simulink model "ECU1119_18b_st"  (R2018b)
settings: Solver=FixedStepDiscrete  StartTime=0.0  StopTime=10.0  RelTol=1e-3
InitFcn:
  | mbd_mpc_consistency_checks(bdroot(gcs));
values from neighbouring files (symbols this model uses):
  ANRtarget = 1.05    [Engine_init.m]
  EGRKi = 0.03    [Engine_init.m]
  EGRKp = 1.2*3    (= 3.6)    [Engine_init.m]
  EGRMax = 1    [Engine_init.m]
  EGRMin = 0    [Engine_init.m]
  EGRTgt = [0.25,0.22,0.20,0.18,0.16,0.12,0.10 ... (first row only)    [Engine_init.m]
  EGRTgt_x = [700,1200,1400,1600,1800,2000,2200]    [Engine_init.m]
  EGRTgt_y = [20,60,100,140,160]    [Engine_init.m]
  EngineSpdTgt = [700:150:2200]    [Engine_init.m]
  EngineSpdTgt_x = [0:10:100]    [Engine_init.m]
  FuelCyleMax = [40,50,60,60,60 ... (first row only)    [Engine_init.m]
  FuelCyleMax_x = [120,180,240,300,360]    [Engine_init.m]
  FuelCyleMax_y = [700,1200,1400,1600,1800,2000,2200]    [Engine_init.m]
  FuelCyleMaxSw = 0    [Engine_init.m]
  FuelCyleMin = 10    [Engine_init.m]
  FuelKd = 0    [Engine_init.m]
  FuelKi = 0.009*5    (= 0.045)    [Engine_init.m]
  FuelKp = 0.03*5    (= 0.15)    [Engine_init.m]
  Regen_Enable_SW = true    [Engine_init.m]
  Soot_Load_Off = 4    [Engine_init.m]
  Soot_Load_On = 18    [Engine_init.m]
  T_regen_max = 680    [Engine_init.m]
  T_regen_min = 550    [Engine_init.m]
undefined symbols (not defined in the file or in its folder): fifo_0_vect, fifo_1_vect, LQFP, pts1_fifo_0_vect, pts1_fifo_1_vect, pts2_fifo_0_vect, pts2_fifo_1_vect, pts3_fifo_0_vect, pts3_fifo_1_vect, pts4_fifo_0_vect, pts4_fifo_1_vect
libraries: mbd_mpc574x_ec_toolbox x111, simulink x12, canmsglib x8
(part 2 of 5)

== system ECU1119_18b_st/ECU ==
  note: 改成%单位了
  EngineSpd_rpm : Inport
  EngineInfo : Inport  Port=2
  ThrottleCmd_pct : Inport  Port=3
  Bus Creator : BusCreator  Inputs=6
  Bus Selector : BusSelector  OutputSignals=Obj_Fast_Fb1 (signal 1).FuelCycle_Act_mg,Obj_Fast_Fb1 (signal 1).EGR_Ratio_Act,Obj_Fast_Fb1 (signal 2).RailPrs_kpa,Obj_Fast_Fb1 (signal 2).IntakeMass_kgph,Obj_Temp_Fb1 (signal 3).DOC_In_Temp_C,Obj_Temp_Fb1 (signal 3).DOC_Out_Temp_C,Obj_Temp_Fb1 (signal 3).DPF_Out_Temp_C,Obj_Temp_Fb2 (signal 4).SCR_Out_Temp_C,Obj_Temp_Fb2 (signal 4).ExhMassFlow_kgph,Obj_Slow_Fb1 (signal 5).NOx_SCR_In_gph,Obj_Slow_Fb1 (signal 5).NOx_SCR_Out_gph,Obj_Slow_Fb1 (signal 5).SootLoad_g,Obj_Slow_Fb1 (signal 5).DPF_dP_kPa,Obj_Slow_Fb2 (signal 6).NH3_Store_g,Obj_Slow_Fb2 (signal 6).O2_frac_pct
  ECU : Subsystem
  Gain{,1..4} (5 alike) : Gain
  EngineCmd : Outport  VectorParamsAs1DForOutWhenUnconnected=on
  wires:
  Bus Selector/13 -> ECU/14(DPF_DP)  "<DPF_dP_kPa>"
  Bus Selector/1 -> ECU/2(FuleCyle_mg)  "<FuelCycle_Act_mg>"
  Bus Selector/14 -> Gain3/1  "<NH3_Store_g>"
  Bus Selector/9 -> ECU/10(ExhMassFlow)  "<ExhMassFlow_kgph>"
  Bus Selector/3 -> ECU/4(RailPrs_kpa)  "<RailPrs_kpa>"
  EngineInfo/1 -> Bus Selector/1
  Bus Selector/10 -> ECU/11(mNOx_SCR_in)  "<NOx_SCR_In_gph>"
  Bus Selector/11 -> Gain2/1  "<NOx_SCR_Out_gph>"
  Bus Selector/12 -> ECU/13(DPF_SootLoad)  "<SootLoad_g>"
  Bus Selector/15 -> Gain4/1  "<O2_frac_pct>"
  Bus Selector/2 -> ECU/3(EGRRatio)  "<EGR_Ratio_Act>"
  Bus Selector/5 -> Gain/1  "<DOC_In_Temp_C>"
  Bus Selector/4 -> ECU/5(IntakeMass)  "<IntakeMass_kgph>"
  Bus Selector/6 -> ECU/7(ExhTemp_DOC_out)  "<DOC_Out_Temp_C>"
  Bus Selector/7 -> ECU/8(ExhTemp_DPF_out)  "<DPF_Out_Temp_C>"
  Bus Selector/8 -> Gain1/1  "<SCR_Out_Temp_C>"
  ECU/3(EGROpeningTgt_pct) -> Bus Creator/3  "EGROpeningTgt_pct"
  ECU/2(FuelCyleTgt_mg) -> Bus Creator/2  "FuelCyleTgt_mg"
  ECU/6(mUREA_target) -> Bus Creator/6  "mUREA_target"
  ECU/1(EngineSpdTgt_rpm) -> Bus Creator/1  "EngineSpdTgt_rpm"
  ECU/5(DPF_regen_req) -> Bus Creator/5  "DPF_regen_req"
  ECU/4(PostInj_Request) -> Bus Creator/4  "PostInj_Request"
  EngineSpd_rpm/1 -> ECU/1(EngineSpd_rpm)
  Bus Creator/1 -> EngineCmd/1
  ThrottleCmd_pct/1 -> ECU/17(ThrottleCmd_pct)
  Gain/1 -> ECU/6(ExhTemp_DOC_in)
  Gain1/1 -> ECU/9(ExhTemp_SCR_out)
  Gain2/1 -> ECU/12(mNOx_SCR_out)
  Gain3/1 -> ECU/15(NH3_Store)
  Gain4/1 -> ECU/16(O2_frac)

== system ECU1119_18b_st/GPIO  ==
  note: LS
  note: PWM
  note: HS
  ETC : Subsystem
  HS : Subsystem
  PWM_OUT : Subsystem  Commented=on
  SPI0: LS09_14_15_16_1_2_11_4 : Subsystem
  SPI3: LS03_06_07_08_10_12_13_17_18_19 : Subsystem

== system ECU1119_18b_st/Init ==
  CAN_init : Subsystem
  Data Store Read1 : DataStoreRead  DataStoreName=VCU_Mode
  Data Store Read3 : DataStoreRead  DataStoreName=Init_flg
  If1 : If  IfExpression=u1 == 2  ShowElse=off
  If2 : If  IfExpression=u1 == 0  ShowElse=off
  Init : Subsystem
  wires:
  Data Store Read3/1 -> If2/1
  If2/1 -> Init/Action
  Data Store Read1/1 -> If1/1
  If1/1 -> CAN_init/Action

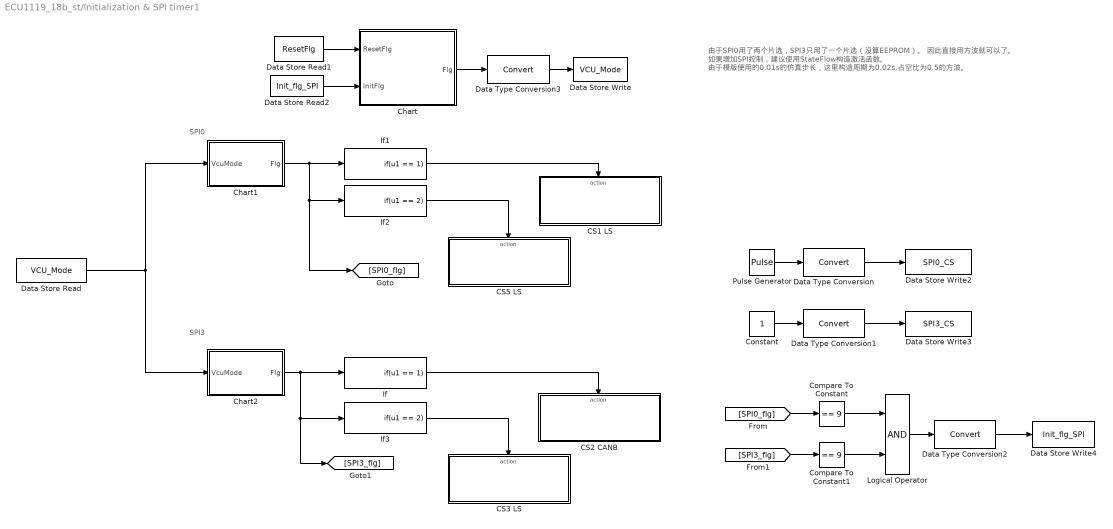
== system ECU1119_18b_st/Initialization & SPI timer1 ==
  note: 由于SPI0用了两个片选，SPI3只用了一个片选（没算EEPROM）。
      | 因此直接用方波就可以了。
      | 如果增加SPI控制，建议使用StateFlow构造激活函数。
      | 由于模版使用的0.01s的仿真步长，这里构造周期为0.02s,占空比为0.5的方波。
  note: SPI3
  note: SPI0
  CS1 LS : Subsystem
  CS2 CANB : Subsystem
  CS3 LS : Subsystem
  CS5 LS : Subsystem
  Chart : Stateflow chart  TreatAsAtomicUnit=on
  Chart1 : Stateflow chart  TreatAsAtomicUnit=on
  Chart2 : Stateflow chart  TreatAsAtomicUnit=on
  Compare To Constant : simulink/Logic and Bit Operations/Compare To Constant  relop===  const=9  OutDataTypeStr=boolean
  Compare To Constant1 : simulink/Logic and Bit Operations/Compare To Constant  relop===  const=9  OutDataTypeStr=boolean
  Constant : Constant
  Data Store Read : DataStoreRead  DataStoreName=VCU_Mode
  Data Store Read1 : DataStoreRead  DataStoreName=ResetFlg
  Data Store Read2 : DataStoreRead  DataStoreName=Init_flg_SPI
  Data Store Write : DataStoreWrite  DataStoreName=VCU_Mode
  Data Store Write2 : DataStoreWrite  DataStoreName=SPI0_CS
  Data Store Write3 : DataStoreWrite  DataStoreName=SPI3_CS
  Data Store Write4 : DataStoreWrite  DataStoreName=Init_flg_SPI
  Data Type Conversion{,1..3} (4 alike) : DataTypeConversion
  If : If  IfExpression=u1 == 1  ShowElse=off
  If1 : If  IfExpression=u1 == 1  ShowElse=off
  If2 : If  IfExpression=u1 == 2  ShowElse=off
  If3 : If  IfExpression=u1 == 2  ShowElse=off
  Logical Operator : Logic  AllPortsSameDT=off  OutDataTypeStr=boolean
  Pulse Generator : DiscretePulseGenerator  PulseType=Time based  Period=0.01  PulseWidth=50
  wires:
  If/1 -> CS2 CANB/Action
  Chart/1(Flg) -> Data Type Conversion3/1
  Data Store Read2/1 -> Chart/2(InitFlg)
  If1/1 -> CS1 LS/Action
  Chart2/1(Flg) -> If3/1, [SPI3_flg], If/1
  Data Store Read/1 -> Chart2/1(VcuMode), Chart1/1(VcuMode)
  If2/1 -> CS5 LS/Action
  [SPI0_flg] -> Compare To Constant/1
  [SPI3_flg] -> Compare To Constant1/1
  Compare To Constant/1 -> Logical Operator/1
  Compare To Constant1/1 -> Logical Operator/2
  Logical Operator/1 -> Data Type Conversion2/1
  If3/1 -> CS3 LS/Action
  Pulse Generator/1 -> Data Type Conversion/1
  Constant/1 -> Data Type Conversion1/1
  Data Type Conversion/1 -> Data Store Write2/1
  Data Type Conversion1/1 -> Data Store Write3/1
  Data Type Conversion2/1 -> Data Store Write4/1
  Data Type Conversion3/1 -> Data Store Write/1
  Chart1/1(Flg) -> If1/1, [SPI0_flg], If2/1
  Data Store Read1/1 -> Chart/1(ResetFlg)

== system ECU1119_18b_st/Power Managment ==
  PowerMode : Inport
  Data Type Conversion : DataTypeConversion
  HS1 : mbd_mpc574x_ec_toolbox/GPIO Blocks/Digital_Output  Priority=1  gpio_pin=PTF6: [SIUL2_GPIO86 | General Purpose IO PF[6]]  gpio_drive_strength=Disabled
      settings: SourceProductName=NXP Model-Based Design Toolbox for MPC57xx MCUs
  HS4 : mbd_mpc574x_ec_toolbox/GPIO Blocks/Digital_Output  Priority=1  gpio_pin=PTA13: [SIUL2_GPIO13 | General Purpose IO PA[13]]  gpio_drive_strength=Disabled
      settings: SourceProductName=NXP Model-Based Design Toolbox for MPC57xx MCUs
  wires:
  PowerMode/1 -> Data Type Conversion/1
  Data Type Conversion/1 -> HS4/1, HS1/1

== system ECU1119_18b_st/SPI_EEPROM ==
  Data Store Memory : DataStoreMemory  DataStoreName=A_write  ReadBeforeWriteMsg=warning  WriteAfterWriteMsg=warning  WriteAfterReadMsg=warning  ShowAdditionalParam=off  OutDataTypeStr=single
      settings: RTWStateStorageClass=ExportedGlobal
  Data Store Memory10 : DataStoreMemory  DataStoreName=A_read  ReadBeforeWriteMsg=warning  WriteAfterWriteMsg=warning  WriteAfterReadMsg=warning  ShowAdditionalParam=off  OutDataTypeStr=single
      settings: RTWStateStorageClass=ExportedGlobal
  Data Store Memory18 : DataStoreMemory  DataStoreName=SPI0_CTRL0  ReadBeforeWriteMsg=warning  WriteAfterWriteMsg=warning  WriteAfterReadMsg=warning  ShowAdditionalParam=off  OutDataTypeStr=uint8
      settings: RTWStateStorageClass=ExportedGlobal
  Data Store Read : DataStoreRead  DataStoreName=SPI0_CTRL0
  SPI_read : Subsystem  TreatAsAtomicUnit=on
  SPI_write : Subsystem  TreatAsAtomicUnit=on
  Switch Case : SwitchCase  CaseConditions={1,2}  ShowDefaultCase=off
  wires:
  Data Store Read/1 -> Switch Case/1
  Switch Case/2 -> SPI_write/Action
  Switch Case/1 -> SPI_read/Action

== system ECU1119_18b_st/SigIn ==
  note: CAN2
  note: HardWareSignalIn
  AI : Subsystem  Commented=on
  CAN0_Rx_500 : mbd_mpc574x_ec_toolbox/Communication Blocks/CAN Blocks/FCAN_Isr  can_instance=2  can_event=Rx Complete
      settings: SourceProductName=NXP Model-Based Design Toolbox for MPC57xx MCUs
  CAN2 : Subsystem  TreatAsAtomicUnit=on
      settings: RTWSystemCode=Nonreusable function
  DI : Subsystem  Commented=on
  PWM : Subsystem  Commented=on
  Terminator : Terminator  Commented=on
  Terminator3 : Terminator  Commented=on
  Terminator5 : Terminator  Commented=on
  Terminator8 : Terminator
  EngineSpd_rpm : Outport  VectorParamsAs1DForOutWhenUnconnected=on
  EngineInfo : Outport  Port=2  VectorParamsAs1DForOutWhenUnconnected=on
  ThrottleCmd_pct : Outport  Port=3  VectorParamsAs1DForOutWhenUnconnected=on
  wires:
  CAN0_Rx_500/5 -> CAN2/3(length)
  CAN0_Rx_500/3 -> CAN2/1(ID)
  CAN0_Rx_500/4 -> CAN2/2(Data)
  CAN0_Rx_500/6 -> CAN2/4(timestamp)
  CAN0_Rx_500/1 -> CAN2/Trigger
  CAN0_Rx_500/2 -> Terminator8/1
  PWM/1(PWMIn) -> Terminator/1
  DI/1(DI) -> Terminator3/1
  AI/1(AI) -> Terminator5/1
  CAN2/3(ThrottleCmd_pct) -> ThrottleCmd_pct/1
  CAN2/2(EngineInfo) -> EngineInfo/1
  CAN2/1(EngineSpd_rpm) -> EngineSpd_rpm/1

== system ECU1119_18b_st/SigOut ==
  note: 10ms
  note: 100ms
  EngCmd : Inport
  Pulse Generator : DiscretePulseGenerator  PulseType=Time based  Period=0.1  PulseWidth=5
  Pulse Generator1 : DiscretePulseGenerator  PulseType=Time based  Period=0.01  PulseWidth=50
  Rate Transition : RateTransition
  Rate Transition1 : RateTransition
  VCU_Cmd_Fast : Subsystem  TreatAsAtomicUnit=on  SystemSampleTime=0.01
  VCU_Cmd_Slow : Subsystem  TreatAsAtomicUnit=on  SystemSampleTime=0.01
  wires:
  EngCmd/1 -> Rate Transition1/1, Rate Transition/1
  Rate Transition/1 -> VCU_Cmd_Fast/1("EngCmd ")
  Pulse Generator1/1 -> VCU_Cmd_Fast/Trigger
  Pulse Generator/1 -> VCU_Cmd_Slow/Trigger
  Rate Transition1/1 -> VCU_Cmd_Slow/1("EngCmd ")

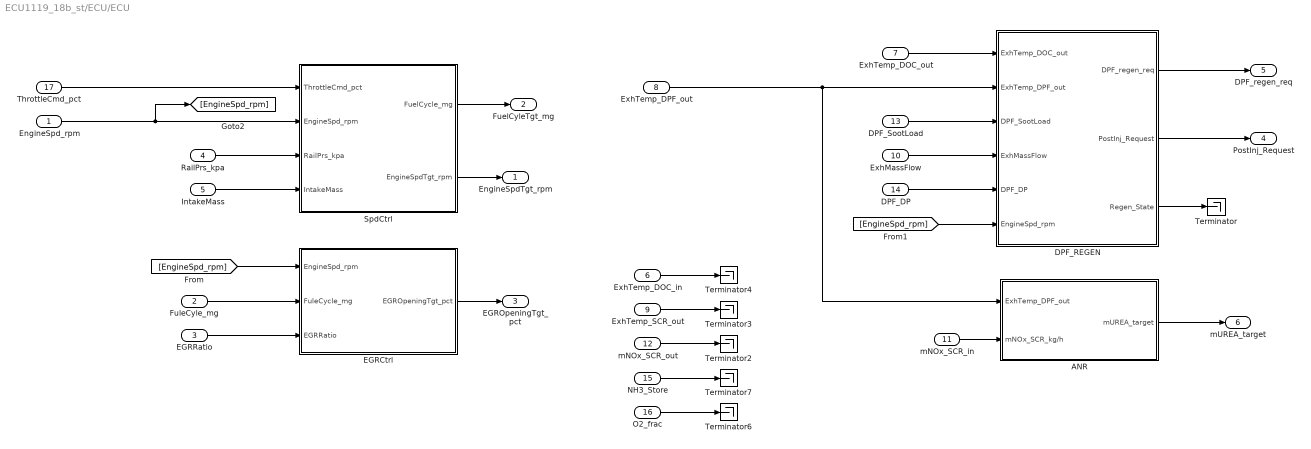
== system ECU1119_18b_st/ECU/ECU ==
  EngineSpd_rpm : Inport
  FuleCyle_mg : Inport  Port=2
  EGRRatio : Inport  Port=3
  RailPrs_kpa : Inport  Port=4
  IntakeMass : Inport  Port=5
  ExhTemp_DOC_in : Inport  Port=6
  ExhTemp_DOC_out : Inport  Port=7
  ExhTemp_DPF_out : Inport  Port=8
  ExhTemp_SCR_out : Inport  Port=9
  ExhMassFlow : Inport  Port=10
  mNOx_SCR_in : Inport  Port=11
  mNOx_SCR_out : Inport  Port=12
  DPF_SootLoad : Inport  Port=13
  DPF_DP : Inport  Port=14
  NH3_Store : Inport  Port=15
  O2_frac : Inport  Port=16
  ThrottleCmd_pct : Inport  Port=17
  ANR : Subsystem
  DPF_REGEN : Subsystem
  EGRCtrl : Subsystem
  SpdCtrl : Subsystem
  Terminator{,2..4,6..7} (6 alike) : Terminator
  EngineSpdTgt_rpm : Outport  VectorParamsAs1DForOutWhenUnconnected=on
  FuelCyleTgt_mg : Outport  Port=2  VectorParamsAs1DForOutWhenUnconnected=on
  EGROpeningTgt_pct : Outport  Port=3  VectorParamsAs1DForOutWhenUnconnected=on
  PostInj_Request : Outport  Port=4  VectorParamsAs1DForOutWhenUnconnected=on
  DPF_regen_req : Outport  Port=5  VectorParamsAs1DForOutWhenUnconnected=on
  mUREA_target : Outport  Port=6  VectorParamsAs1DForOutWhenUnconnected=on
  wires:
  SpdCtrl/1(FuelCycle_mg) -> FuelCyleTgt_mg/1
  EngineSpd_rpm/1 -> [EngineSpd_rpm], SpdCtrl/2(EngineSpd_rpm)
  FuleCyle_mg/1 -> EGRCtrl/2(FuleCycle_mg)
  EGRCtrl/1(EGROpeningTgt_pct) -> EGROpeningTgt_pct/1
  EGRRatio/1 -> EGRCtrl/3(EGRRatio)
  RailPrs_kpa/1 -> SpdCtrl/3(RailPrs_kpa)
  IntakeMass/1 -> SpdCtrl/4(IntakeMass)
  [EngineSpd_rpm] -> EGRCtrl/1(EngineSpd_rpm)
  mNOx_SCR_in/1 -> ANR/2(mNOx_SCR_kg/h)
  ANR/1(mUREA_target) -> mUREA_target/1
  ExhTemp_DPF_out/1 -> DPF_REGEN/2(ExhTemp_DPF_out), ANR/1(ExhTemp_DPF_out)
  DPF_SootLoad/1 -> DPF_REGEN/3(DPF_SootLoad)
  ExhMassFlow/1 -> DPF_REGEN/4(ExhMassFlow)
  DPF_REGEN/1(DPF_regen_req) -> DPF_regen_req/1
  ExhTemp_DOC_in/1 -> Terminator4/1
  mNOx_SCR_out/1 -> Terminator2/1
  ExhTemp_SCR_out/1 -> Terminator3/1
  NH3_Store/1 -> Terminator7/1
  O2_frac/1 -> Terminator6/1
  DPF_DP/1 -> DPF_REGEN/5(DPF_DP)
  ExhTemp_DOC_out/1 -> DPF_REGEN/1(ExhTemp_DOC_out)
  [EngineSpd_rpm] -> DPF_REGEN/6(EngineSpd_rpm)
  DPF_REGEN/2(PostInj_Request) -> PostInj_Request/1
  ThrottleCmd_pct/1 -> SpdCtrl/1(ThrottleCmd_pct)
  SpdCtrl/2(EngineSpdTgt_rpm) -> EngineSpdTgt_rpm/1
  DPF_REGEN/3(Regen_State) -> Terminator/1

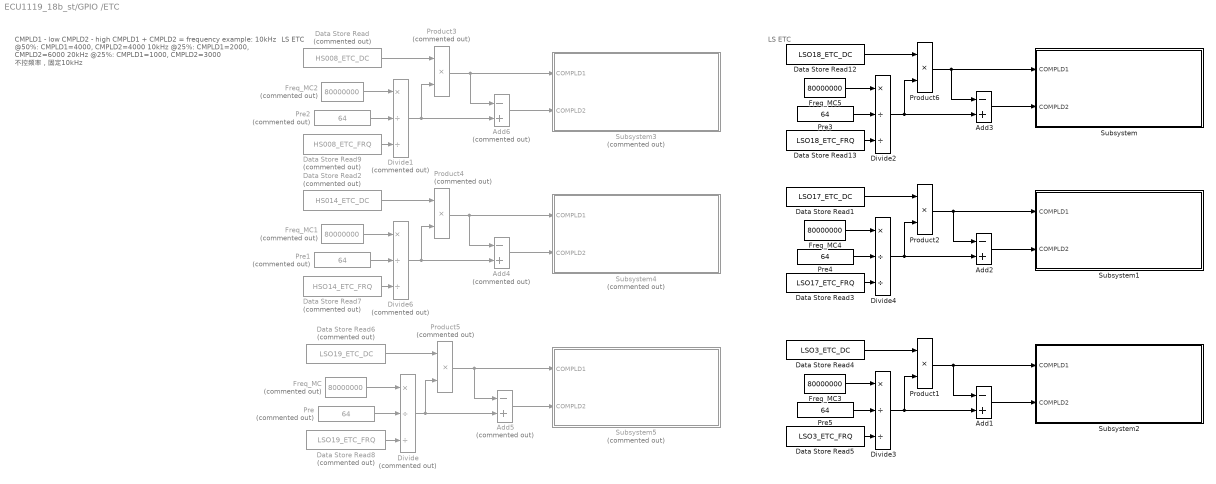
== system ECU1119_18b_st/GPIO /ETC ==
  note: CMPLD1 - low
      | CMPLD2 - high
      | CMPLD1 + CMPLD2 = frequency
      | example:
      | 10kHz @50%: CMPLD1=4000, CMPLD2=4000
      | 10kHz @25%: CMPLD1=2000, CMPLD2=6000
      | 20kHz @25%: CMPLD1=1000, CMPLD2=3000
      |
      | 不控频率，固定10kHz
  note: LS ETC
  note: LS ETC
  Add1 : Sum  Inputs=-+
  Add2 : Sum  Inputs=-+
  Add3 : Sum  Inputs=-+
  Add4 : Sum  Commented=on  Inputs=-+
  Add5 : Sum  Commented=on  Inputs=-+
  Add6 : Sum  Commented=on  Inputs=-+
  Data Store Read : DataStoreRead  Commented=on  DataStoreName=HS008_ETC_DC
  Data Store Read1 : DataStoreRead  DataStoreName=LSO17_ETC_DC
  Data Store Read12 : DataStoreRead  DataStoreName=LSO18_ETC_DC
  Data Store Read13 : DataStoreRead  DataStoreName=LSO18_ETC_FRQ
  Data Store Read2 : DataStoreRead  Commented=on  DataStoreName=HS014_ETC_DC
  Data Store Read3 : DataStoreRead  DataStoreName=LSO17_ETC_FRQ
  Data Store Read4 : DataStoreRead  DataStoreName=LSO3_ETC_DC
  Data Store Read5 : DataStoreRead  DataStoreName=LSO3_ETC_FRQ
  Data Store Read6 : DataStoreRead  Commented=on  DataStoreName=LSO19_ETC_DC
  Data Store Read7 : DataStoreRead  Commented=on  DataStoreName=HSO14_ETC_FRQ
  Data Store Read8 : DataStoreRead  Commented=on  DataStoreName=LSO19_ETC_FRQ
  Data Store Read9 : DataStoreRead  Commented=on  DataStoreName=HS008_ETC_FRQ
  Divide : Product  Commented=on  Inputs=*//
  Divide1 : Product  Commented=on  Inputs=*//
  Divide2 : Product  Inputs=*//
  Divide3 : Product  Inputs=*//
  Divide4 : Product  Inputs=*//
  Divide6 : Product  Commented=on  Inputs=*//
  Freq_MC : Constant  Commented=on  Value=80000000  OutDataTypeStr=single
  Freq_MC1 : Constant  Commented=on  Value=80000000  OutDataTypeStr=single
  Freq_MC2 : Constant  Commented=on  Value=80000000  OutDataTypeStr=single
  Freq_MC3 : Constant  Value=80000000  OutDataTypeStr=single
  Freq_MC4 : Constant  Value=80000000  OutDataTypeStr=single
  Freq_MC5 : Constant  Value=80000000  OutDataTypeStr=single
  Pre : Constant  Commented=on  Value=64
  Pre1 : Constant  Commented=on  Value=64
  Pre2 : Constant  Commented=on  Value=64
  Pre3 : Constant  Value=64
  Pre4 : Constant  Value=64
  Pre5 : Constant  Value=64
  Product1 : Product
  Product2 : Product
  Product3 : Product  Commented=on
  Product4 : Product  Commented=on
  Product5 : Product  Commented=on
  Product6 : Product
  Subsystem : Subsystem
  Subsystem1 : Subsystem
  Subsystem2 : Subsystem
  Subsystem3 : Subsystem  Commented=on
  Subsystem4 : Subsystem  Commented=on
  Subsystem5 : Subsystem  Commented=on
  wires:
  Data Store Read6/1 -> Product5/1
  Product5/1 -> Add5/1, Subsystem5/1(COMPLD1)
  Add5/1 -> Subsystem5/2(COMPLD2)
  Add4/1 -> Subsystem4/2(COMPLD2)
  Data Store Read8/1 -> Divide/3
  Data Store Read2/1 -> Product4/1
  Freq_MC/1 -> Divide/1
  Divide/1 -> Product5/2, Add5/2
  Divide6/1 -> Product4/2, Add4/2
  Freq_MC1/1 -> Divide6/1
  Data Store Read7/1 -> Divide6/3
  Product4/1 -> Add4/1, Subsystem4/1(COMPLD1)
  Divide1/1 -> Product3/2, Add6/2
  Freq_MC2/1 -> Divide1/1
  Data Store Read9/1 -> Divide1/3
  Product3/1 -> Add6/1, Subsystem3/1(COMPLD1)
  Data Store Read/1 -> Product3/1
  Add6/1 -> Subsystem3/2(COMPLD2)
  Divide3/1 -> Product1/2, Add1/2
  Freq_MC3/1 -> Divide3/1
  Data Store Read5/1 -> Divide3/3
  Product1/1 -> Add1/1, Subsystem2/1(COMPLD1)
  Divide4/1 -> Product2/2, Add2/2
  Freq_MC4/1 -> Divide4/1
  Data Store Read3/1 -> Divide4/3
  Product2/1 -> Add2/1, Subsystem1/1(COMPLD1)
  Divide2/1 -> Product6/2, Add3/2
  Freq_MC5/1 -> Divide2/1
  Data Store Read13/1 -> Divide2/3
  Product6/1 -> Add3/1, Subsystem/1(COMPLD1)
  Data Store Read1/1 -> Product2/1
  Data Store Read4/1 -> Product1/1
  Data Store Read12/1 -> Product6/1
  Add1/1 -> Subsystem2/2(COMPLD2)
  Add2/1 -> Subsystem1/2(COMPLD2)
  Add3/1 -> Subsystem/2(COMPLD2)
  Pre/1 -> Divide/2
  Pre1/1 -> Divide6/2
  Pre2/1 -> Divide1/2
  Pre3/1 -> Divide2/2
  Pre4/1 -> Divide4/2
  Pre5/1 -> Divide3/2

== system ECU1119_18b_st/GPIO /HS ==
  note: 3A/5A
  note: 1A/3A
  note: 0.5A/1A
  Data Store Read : DataStoreRead  DataStoreName=HS001
  Data Store Read2 : DataStoreRead  DataStoreName=HS007
  Data Store Read4 : DataStoreRead  DataStoreName=HS002
  Data Store Read5 : DataStoreRead  DataStoreName=HS003
  Data Store Read6 : DataStoreRead  DataStoreName=HS004
  Data Store Read7 : DataStoreRead  DataStoreName=HS005
  Data Store Read9 : DataStoreRead  DataStoreName=HS010
  HS001 : mbd_mpc574x_ec_toolbox/GPIO Blocks/Digital_Output  Priority=1  gpio_pin=PTF5: [SIUL2_GPIO85 | General Purpose IO PF[5]]  gpio_drive_strength=Disabled
      settings: SourceProductName=NXP Model-Based Design Toolbox for MPC57xx MCUs
  "HS002 " : mbd_mpc574x_ec_toolbox/GPIO Blocks/Digital_Output  Priority=1  gpio_pin=PTF4: [SIUL2_GPIO84 | General Purpose IO PF[4]]  gpio_drive_strength=Disabled
      settings: SourceProductName=NXP Model-Based Design Toolbox for MPC57xx MCUs
  HS003 : mbd_mpc574x_ec_toolbox/GPIO Blocks/Digital_Output  Priority=1  gpio_pin=PTF3: [SIUL2_GPIO83 | General Purpose IO PF[3]]  gpio_drive_strength=Disabled
      settings: SourceProductName=NXP Model-Based Design Toolbox for MPC57xx MCUs
  HS004 : mbd_mpc574x_ec_toolbox/GPIO Blocks/Digital_Output  Priority=1  gpio_pin=PTB6: [SIUL2_GPIO22 | General Purpose IO PB[6]]  gpio_drive_strength=Disabled
      settings: SourceProductName=NXP Model-Based Design Toolbox for MPC57xx MCUs
  HS005 : mbd_mpc574x_ec_toolbox/GPIO Blocks/Digital_Output  Priority=1  gpio_pin=PTA12: [SIUL2_GPIO12 | General Purpose IO PA[12]]  gpio_drive_strength=Disabled
      settings: SourceProductName=NXP Model-Based Design Toolbox for MPC57xx MCUs
  HS007 : mbd_mpc574x_ec_toolbox/GPIO Blocks/Digital_Output  Priority=1  gpio_pin=PTF7: [SIUL2_GPIO87 | General Purpose IO PF[7]]  gpio_drive_strength=Disabled
      settings: SourceProductName=NXP Model-Based Design Toolbox for MPC57xx MCUs
  HS010 : mbd_mpc574x_ec_toolbox/GPIO Blocks/Digital_Output  Priority=1  gpio_pin=PTF9: [SIUL2_GPIO89 | General Purpose IO PF[9]]  gpio_drive_strength=Disabled
      settings: SourceProductName=NXP Model-Based Design Toolbox for MPC57xx MCUs
  wires:
  Data Store Read/1 -> HS001/1
  Data Store Read5/1 -> HS003/1
  Data Store Read4/1 -> "HS002 "/1
  Data Store Read6/1 -> HS004/1
  Data Store Read7/1 -> HS005/1
  Data Store Read2/1 -> HS007/1
  Data Store Read9/1 -> HS010/1

== system ECU1119_18b_st/GPIO /PWM_OUT ==
  note: LS PWM
  note: HS PWM
  note: Example
  Data Store Read10 : DataStoreRead  DataStoreName=HSO14_PWM_DC
  Data Store Read11 : DataStoreRead  DataStoreName=HSO14_PWM_FRQ
  Data Store Read14 : DataStoreRead  DataStoreName=LSO19_PWM_DC
  Data Store Read15 : DataStoreRead  DataStoreName=LSO19_PWM_FRQ
  Data Store Read2 : DataStoreRead  DataStoreName=HSO08_PWM_DC
  Data Store Read9 : DataStoreRead  DataStoreName=HSO08_PWM_FRQ
  FreqCMD : Stateflow chart  Priority=0  Commented=on  TreatAsAtomicUnit=on
  PWM Configuration and Frequency Update : Subsystem  Commented=on
  PWM Configuration and Frequency Update1 : Subsystem
  PWM Configuration and Frequency Update4 : Subsystem
  wires:
  FreqCMD/1(freq) -> PWM Configuration and Frequency Update/1(In1)
  FreqCMD/2(dc) -> PWM Configuration and Frequency Update/2(In2)
  Data Store Read9/1 -> PWM Configuration and Frequency Update1/2(Fre A)
  Data Store Read2/1 -> PWM Configuration and Frequency Update1/1(PWM A)
  Data Store Read14/1 -> PWM Configuration and Frequency Update4/1(PWM A)
  Data Store Read10/1 -> PWM Configuration and Frequency Update1/3(PWM B)
  Data Store Read11/1 -> PWM Configuration and Frequency Update1/4(Fre B)
  Data Store Read15/1 -> PWM Configuration and Frequency Update4/2(Fre)

== system ECU1119_18b_st/GPIO /SPI0: LS09_14_15_16_1_2_11_4 ==
  note: 不要开，会重置SPI的初始化设置
  Compare To Constant : simulink/Logic and Bit Operations/Compare To Constant  relop===  const=2  OutDataTypeStr=boolean
  Constant : Constant  OutDataTypeStr=boolean
  Constant1 : Constant  OutDataTypeStr=boolean
  Constant2 : Constant  OutDataTypeStr=boolean
  Data Store Read : DataStoreRead  DataStoreName=VCU_Mode
  Data Store Read1 : DataStoreRead  DataStoreName=SPI0_CS
  LS_CTRL : Subsystem
  LS_CTRL1 : Subsystem
  LS_EN : mbd_mpc574x_ec_toolbox/GPIO Blocks/Digital_Output  Priority=1  gpio_pin=PTA2: [SIUL2_GPIO2 | General Purpose IO PA[2]]  gpio_drive_strength=Disabled
      settings: SourceProductName=NXP Model-Based Design Toolbox for MPC57xx MCUs
  LS_rst1 : mbd_mpc574x_ec_toolbox/GPIO Blocks/Digital_Output  Priority=1  gpio_pin=PTC10: [SIUL2_GPIO42 | General Purpose IO PC[10]]  gpio_drive_strength=Disabled
      settings: SourceProductName=NXP Model-Based Design Toolbox for MPC57xx MCUs
  LS_rst2 : mbd_mpc574x_ec_toolbox/GPIO Blocks/Digital_Output  Priority=1  gpio_pin=PTA1: [SIUL2_GPIO1 | General Purpose IO PA[1]]  gpio_drive_strength=Disabled
      settings: SourceProductName=NXP Model-Based Design Toolbox for MPC57xx MCUs
  Logical Operator : Logic  AllPortsSameDT=off  OutDataTypeStr=boolean
  Logical Operator1 : Logic  Operator=NOT  AllPortsSameDT=off  OutDataTypeStr=boolean
  wires:
  Constant1/1 -> LS_rst2/1
  Constant/1 -> LS_EN/1
  Constant2/1 -> LS_rst1/1
  Data Store Read/1 -> Compare To Constant/1
  Compare To Constant/1 -> Logical Operator/1
  Data Store Read1/1 -> Logical Operator/2
  Logical Operator/1 -> LS_CTRL1/Enable, Logical Operator1/1
  Logical Operator1/1 -> LS_CTRL/Enable

== system ECU1119_18b_st/GPIO /SPI3: LS03_06_07_08_10_12_13_17_18_19 ==
  Compare To Constant : simulink/Logic and Bit Operations/Compare To Constant  relop===  const=2  OutDataTypeStr=boolean
  Constant1 : Constant  OutDataTypeStr=boolean
  Constant3 : Constant  OutDataTypeStr=boolean
  Data Store Read : DataStoreRead  DataStoreName=VCU_Mode
  Data Store Read3 : DataStoreRead  DataStoreName=SPI3_CS
  LS_EN1 : mbd_mpc574x_ec_toolbox/GPIO Blocks/Digital_Output  Priority=1  gpio_pin=PTF10: [SIUL2_GPIO90 | General Purpose IO PF[10]]  gpio_drive_strength=Disabled
      settings: SourceProductName=NXP Model-Based Design Toolbox for MPC57xx MCUs
  LS_rst : mbd_mpc574x_ec_toolbox/GPIO Blocks/Digital_Output  Priority=1  gpio_pin=PTC14: [SIUL2_GPIO46 | General Purpose IO PC[14]]  gpio_drive_strength=Disabled
      settings: SourceProductName=NXP Model-Based Design Toolbox for MPC57xx MCUs
  Logical Operator : Logic  AllPortsSameDT=off  OutDataTypeStr=boolean
  Subsystem : Subsystem
  wires:
  Constant1/1 -> LS_EN1/1
  Constant3/1 -> LS_rst/1
  Data Store Read/1 -> Compare To Constant/1
  Data Store Read3/1 -> Logical Operator/2
  Compare To Constant/1 -> Logical Operator/1
  Logical Operator/1 -> Subsystem/Enable

== system ECU1119_18b_st/Init/CAN_init ==
  note: CAN2
  Action Port : ActionPort  ActionType=then
  Obj_Fast_Fb1 : mbd_mpc574x_ec_toolbox/Communication Blocks/CAN Blocks/FCAN_Receive  can_instance=2  can_mode=Non-blocking  can_timeout_ms=0  can_mb_idx=0  can_extended_id=off  can_is_remote=off  can_id=101  can_msg_mask=FFFFFFFF  show_adv_opts=off  can_use_rxfifo=off  can_fd_enable=off
      settings: SourceProductName=NXP Model-Based Design Toolbox for MPC57xx MCUs
  Obj_Fast_Fb2 : mbd_mpc574x_ec_toolbox/Communication Blocks/CAN Blocks/FCAN_Receive  can_instance=2  can_mode=Non-blocking  can_timeout_ms=0  can_mb_idx=1  can_extended_id=off  can_is_remote=off  can_id=102  can_msg_mask=FFFFFFFF  show_adv_opts=off  can_use_rxfifo=off  can_fd_enable=off
      settings: SourceProductName=NXP Model-Based Design Toolbox for MPC57xx MCUs
  Obj_Slow_Fb1 : mbd_mpc574x_ec_toolbox/Communication Blocks/CAN Blocks/FCAN_Receive  can_instance=2  can_mode=Non-blocking  can_timeout_ms=0  can_mb_idx=4  can_extended_id=off  can_is_remote=off  can_id=105  can_msg_mask=FFFFFFFF  show_adv_opts=off  can_use_rxfifo=off  can_fd_enable=off
      settings: SourceProductName=NXP Model-Based Design Toolbox for MPC57xx MCUs
  Obj_Slow_Fb2 : mbd_mpc574x_ec_toolbox/Communication Blocks/CAN Blocks/FCAN_Receive  can_instance=2  can_mode=Non-blocking  can_timeout_ms=0  can_mb_idx=5  can_extended_id=off  can_is_remote=off  can_id=106  can_msg_mask=FFFFFFFF  show_adv_opts=off  can_use_rxfifo=off  can_fd_enable=off
      settings: SourceProductName=NXP Model-Based Design Toolbox for MPC57xx MCUs
  Obj_Temp_Fb1 : mbd_mpc574x_ec_toolbox/Communication Blocks/CAN Blocks/FCAN_Receive  can_instance=2  can_mode=Non-blocking  can_timeout_ms=0  can_mb_idx=2  can_extended_id=off  can_is_remote=off  can_id=103  can_msg_mask=FFFFFFFF  show_adv_opts=off  can_use_rxfifo=off  can_fd_enable=off
      settings: SourceProductName=NXP Model-Based Design Toolbox for MPC57xx MCUs
  Obj_Temp_Fb2 : mbd_mpc574x_ec_toolbox/Communication Blocks/CAN Blocks/FCAN_Receive  can_instance=2  can_mode=Non-blocking  can_timeout_ms=0  can_mb_idx=3  can_extended_id=off  can_is_remote=off  can_id=104  can_msg_mask=FFFFFFFF  show_adv_opts=off  can_use_rxfifo=off  can_fd_enable=off
      settings: SourceProductName=NXP Model-Based Design Toolbox for MPC57xx MCUs

== system ECU1119_18b_st/Init/Init ==
  note: MainRelay
  Action Port : ActionPort  ActionType=then
  Chart : Stateflow chart  TreatAsAtomicUnit=on
  Constant : Constant
  Data Store Read1 : DataStoreRead  DataStoreName=KeyOn
  Data Store Write : DataStoreWrite  DataStoreName=LS001
  Data Store Write3 : DataStoreWrite  DataStoreName=Init_flg
  Data Type Conversion : DataTypeConversion
  Data Type Conversion1 : DataTypeConversion  OutDataTypeStr=boolean
  wires:
  Constant/1 -> Data Type Conversion/1
  Data Type Conversion/1 -> Data Store Write3/1
  Chart/1(LS001) -> Data Type Conversion1/1
  Data Store Read1/1 -> Chart/1(KeyOn)
  Data Type Conversion1/1 -> Data Store Write/1

== system ECU1119_18b_st/Initialization & SPI timer1/CS1 LS ==
  Action Port : ActionPort  ActionType=then
  Chart : Stateflow chart  TreatAsAtomicUnit=on
  Data Type Conversion{,1,3..4} (4 alike) : DataTypeConversion
  Demux1 : Demux  Outputs=2
  SPI_Master_Transfer_To1 : mbd_mpc574x_ec_toolbox/Communication Blocks/SPI Blocks/SPI_Master_Transfer  Priority=2  InstanceNumber=0  xfermode=Non blocking  timeout=50  spi_upd=on  WhichPCS=5
      settings: SourceProductName=NXP Model-Based Design Toolbox for MPC57xx MCUs
  Subsystem : Subsystem  Commented=on
  Terminator : Terminator
  Terminator1 : Terminator
  Vector Concatenate1 : Concatenate
  wires:
  SPI_Master_Transfer_To1/1 -> Demux1/1
  Data Type Conversion3/1 -> Terminator/1
  Vector Concatenate1/1 -> SPI_Master_Transfer_To1/1
  Demux1/2 -> Data Type Conversion4/1
  Data Type Conversion4/1 -> Terminator1/1
  Demux1/1 -> Data Type Conversion3/1
  Chart/1(high) -> Data Type Conversion/1
  Chart/2(low) -> Data Type Conversion1/1
  Data Type Conversion/1 -> Vector Concatenate1/1
  Data Type Conversion1/1 -> Vector Concatenate1/2

== system ECU1119_18b_st/Initialization & SPI timer1/CS2 CANB ==
  Action Port : ActionPort  ActionType=then
  Constant : Constant  Value=2
  Constant1 : Constant  Value=7
  Data Type Conversion : DataTypeConversion  OutDataTypeStr=uint8
  Data Type Conversion1 : DataTypeConversion  OutDataTypeStr=uint8
  Data Type Conversion2 : DataTypeConversion
  Data Type Conversion3 : DataTypeConversion
  Demux2 : Demux  Outputs=2
  SPI_Master_Transfer_To2 : mbd_mpc574x_ec_toolbox/Communication Blocks/SPI Blocks/SPI_Master_Transfer  Priority=2  InstanceNumber=3  xfermode=Non blocking  timeout=50  spi_upd=on  WhichPCS=2
      settings: SourceProductName=NXP Model-Based Design Toolbox for MPC57xx MCUs
  Terminator : Terminator
  Terminator1 : Terminator
  Vector Concatenate2 : Concatenate
  wires:
  Vector Concatenate2/1 -> SPI_Master_Transfer_To2/1
  Demux2/2 -> Data Type Conversion1/1
  Data Type Conversion2/1 -> Vector Concatenate2/2
  SPI_Master_Transfer_To2/1 -> Demux2/1
  Data Type Conversion1/1 -> Terminator1/1
  Data Type Conversion/1 -> Terminator/1
  Demux2/1 -> Data Type Conversion/1
  Data Type Conversion3/1 -> Vector Concatenate2/1
  Constant/1 -> Data Type Conversion3/1
  Constant1/1 -> Data Type Conversion2/1

== system ECU1119_18b_st/Initialization & SPI timer1/CS3 LS ==
  note: 80-0101 0000 - 对A组端口控制模式进行设置
      | 96-0110 0000 - 对B组端口控制模式进行设置
      | 40-0010 1100 -使用SPI控制端口
      |
      | 其中端口1,2,5,6即为复用PWM端口，这里设置为引脚控制（A组），其余端口设置为SPI控制
  Action Port : ActionPort  ActionType=then
  Chart : Stateflow chart  TreatAsAtomicUnit=on
  Data Type Conversion : DataTypeConversion  OutDataTypeStr=uint8
  Data Type Conversion1 : DataTypeConversion  OutDataTypeStr=uint8
  Data Type Conversion2 : DataTypeConversion
  Data Type Conversion3 : DataTypeConversion
  Demux2 : Demux  Outputs=2
  Manual Switch : ManualSwitch  CurrentSetting=0
  PIN : Constant  Value=2
  SPI : Constant  Value=0
  SPI_Master_Transfer_To2 : mbd_mpc574x_ec_toolbox/Communication Blocks/SPI Blocks/SPI_Master_Transfer  Priority=2  InstanceNumber=3  xfermode=Non blocking  timeout=50  spi_upd=on  WhichPCS=3
      settings: SourceProductName=NXP Model-Based Design Toolbox for MPC57xx MCUs
  Subsystem : Subsystem  Commented=on
  Terminator2 : Terminator
  Terminator3 : Terminator
  Vector Concatenate1 : Concatenate
  wires:
  Data Type Conversion1/1 -> Terminator3/1
  Data Type Conversion/1 -> Terminator2/1
  Demux2/1 -> Data Type Conversion/1
  SPI_Master_Transfer_To2/1 -> Demux2/1
  Demux2/2 -> Data Type Conversion1/1
  Chart/2(low) -> Data Type Conversion3/1
  Vector Concatenate1/1 -> SPI_Master_Transfer_To2/1
  Data Type Conversion2/1 -> Vector Concatenate1/1
  Data Type Conversion3/1 -> Vector Concatenate1/2
  Chart/1(high) -> Data Type Conversion2/1
  PIN/1 -> Manual Switch/2
  SPI/1 -> Manual Switch/1
  Manual Switch/1 -> [Mode]
  [Mode] -> Chart/1(mode)

== system ECU1119_18b_st/Initialization & SPI timer1/CS5 LS ==
  Action Port : ActionPort  ActionType=then
  Chart : Stateflow chart  TreatAsAtomicUnit=on
  Data Type Conversion{,1,3..4} (4 alike) : DataTypeConversion
  Demux1 : Demux  Outputs=2
  SPI_Master_Transfer_To1 : mbd_mpc574x_ec_toolbox/Communication Blocks/SPI Blocks/SPI_Master_Transfer  Priority=2  InstanceNumber=0  xfermode=Non blocking  timeout=50  spi_upd=on  WhichPCS=1
      settings: SourceProductName=NXP Model-Based Design Toolbox for MPC57xx MCUs
  Subsystem : Subsystem  Commented=on
  Terminator : Terminator
  Terminator1 : Terminator
  Vector Concatenate1 : Concatenate
  wires:
  SPI_Master_Transfer_To1/1 -> Demux1/1
  Demux1/1 -> Data Type Conversion3/1
  Data Type Conversion3/1 -> Terminator/1
  Demux1/2 -> Data Type Conversion4/1
  Data Type Conversion4/1 -> Terminator1/1
  Chart/2(low) -> Data Type Conversion1/1
  Vector Concatenate1/1 -> SPI_Master_Transfer_To1/1
  Data Type Conversion/1 -> Vector Concatenate1/1
  Data Type Conversion1/1 -> Vector Concatenate1/2
  Chart/1(high) -> Data Type Conversion/1

== system ECU1119_18b_st/SPI_EEPROM/SPI_read ==
  Action Port : ActionPort
  "Address_High " : Constant  Value=hex2dec('FF')  OutDataTypeStr=uint8
  Address_Low : Constant  Value=hex2dec('FF')
  Bitwise AND : simulink/Logic and Bit Operations/Bitwise Operator  logicop=AND  UseBitMask=on  BitMask=hex2dec('00FF')  BitMaskRealWorld=Stored Integer
  Constant : Constant  Value=0
  Data Store Write : DataStoreWrite  DataStoreName=A_read
  Data Type Conversion{,1,3..8} (8 alike) : DataTypeConversion  OutDataTypeStr=uint8
  Data Type Conversion2 : DataTypeConversion
  Demux1 : Demux
  SPI_Master_Transfer_To1 : mbd_mpc574x_ec_toolbox/Communication Blocks/SPI Blocks/SPI_Master_Transfer  Priority=2  InstanceNumber=0  xfermode=Non blocking  timeout=50  spi_upd=on  WhichPCS=0
      settings: SourceProductName=NXP Model-Based Design Toolbox for MPC57xx MCUs
  Terminator : Terminator
  Terminator1 : Terminator
  Terminator2 : Terminator
  Vector Concatenate1 : Concatenate  NumInputs=4
  read_set : Constant  Value=3  OutDataTypeStr=uint8
  wires:
  "Address_High "/1 -> Data Type Conversion1/1
  read_set/1 -> Data Type Conversion/1
  Data Type Conversion1/1 -> Vector Concatenate1/2  "d1"
  Data Type Conversion/1 -> Vector Concatenate1/1  "d0"
  Address_Low/1 -> Data Type Conversion6/1
  Demux1/2 -> Data Type Conversion4/1
  Vector Concatenate1/1 -> SPI_Master_Transfer_To1/1
  Demux1/1 -> Data Type Conversion3/1
  SPI_Master_Transfer_To1/1 -> Demux1/1
  Data Type Conversion3/1 -> Terminator/1  "r0"
  Data Type Conversion8/1 -> Bitwise AND/1  "r3"
  Bitwise AND/1 -> Data Type Conversion2/1
  Data Type Conversion2/1 -> Data Store Write/1
  Constant/1 -> Data Type Conversion7/1
  Data Type Conversion6/1 -> Vector Concatenate1/3  "d2"
  Data Type Conversion7/1 -> Vector Concatenate1/4  "d3"
  Demux1/3 -> Data Type Conversion5/1
  Data Type Conversion4/1 -> Terminator1/1  "r1"
  Data Type Conversion5/1 -> Terminator2/1  "r2"
  Demux1/4 -> Data Type Conversion8/1

== system ECU1119_18b_st/SPI_EEPROM/SPI_write ==
  Action Port : ActionPort
  Data Store Memory : DataStoreMemory  DataStoreName=Write_Ctrl  ReadBeforeWriteMsg=warning  WriteAfterWriteMsg=warning  WriteAfterReadMsg=warning  InitialValue=1  ShowAdditionalParam=off  OutDataTypeStr=uint8
      settings: RTWStateStorageClass=ExportedGlobal
  Data Store Read : DataStoreRead  DataStoreName=Write_Ctrl
  SPI_enable : Subsystem  TreatAsAtomicUnit=on
  SPI_write : Subsystem  TreatAsAtomicUnit=on
  Switch Case : SwitchCase  CaseConditions={1,2}  ShowDefaultCase=off
  wires:
  Data Store Read/1 -> Switch Case/1
  Switch Case/2 -> SPI_write/Action
  Switch Case/1 -> SPI_enable/Action

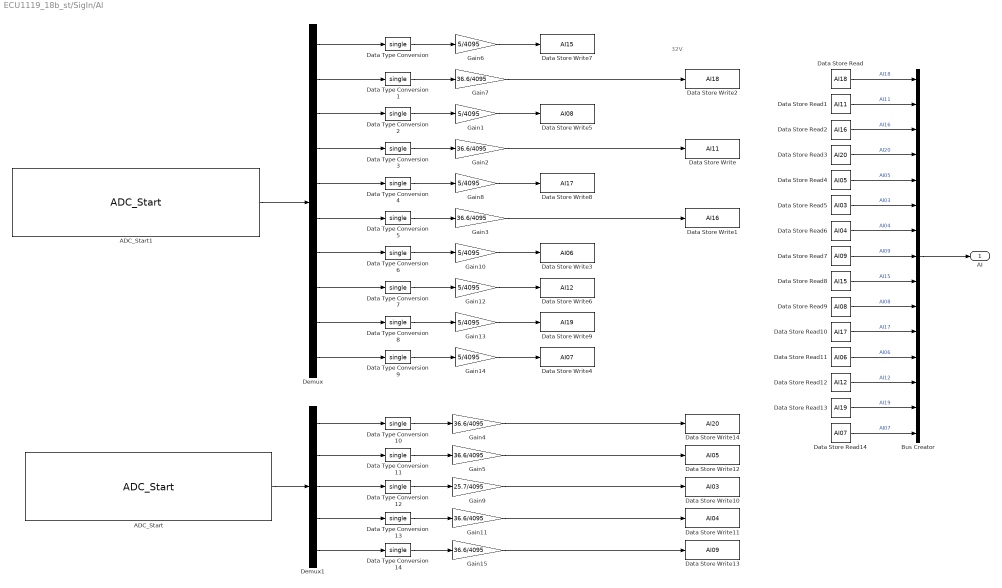
== system ECU1119_18b_st/SigIn/AI ==
  note: 32V
  ADC_Start : mbd_mpc574x_ec_toolbox/Motor Control Blocks/ADC Blocks/ADC_Start  adc_instance=1  interrupt=off  presample=off
      settings: SourceProductName=NXP Model-Based Design Toolbox for MPC57xx MCUs
  ADC_Start1 : mbd_mpc574x_ec_toolbox/Motor Control Blocks/ADC Blocks/ADC_Start  adc_instance=0  interrupt=off  presample=off
      settings: SourceProductName=NXP Model-Based Design Toolbox for MPC57xx MCUs
  Bus Creator : BusCreator  Inputs=15
  Data Store Read : DataStoreRead  DataStoreName=AI18
  Data Store Read1 : DataStoreRead  DataStoreName=AI11
  Data Store Read10 : DataStoreRead  DataStoreName=AI17
  Data Store Read11 : DataStoreRead  DataStoreName=AI06
  Data Store Read12 : DataStoreRead  DataStoreName=AI12
  Data Store Read13 : DataStoreRead  DataStoreName=AI19
  Data Store Read14 : DataStoreRead  DataStoreName=AI07
  Data Store Read2 : DataStoreRead  DataStoreName=AI16
  Data Store Read3 : DataStoreRead  DataStoreName=AI20
  Data Store Read4 : DataStoreRead  DataStoreName=AI05
  Data Store Read5 : DataStoreRead  DataStoreName=AI03
  Data Store Read6 : DataStoreRead  DataStoreName=AI04
  Data Store Read7 : DataStoreRead  DataStoreName=AI09
  Data Store Read8 : DataStoreRead  DataStoreName=AI15
  Data Store Read9 : DataStoreRead  DataStoreName=AI08
  Data Store Write : DataStoreWrite  DataStoreName=AI11
  Data Store Write1 : DataStoreWrite  DataStoreName=AI16
  Data Store Write10 : DataStoreWrite  DataStoreName=AI03
  Data Store Write11 : DataStoreWrite  DataStoreName=AI04
  Data Store Write12 : DataStoreWrite  DataStoreName=AI05
  Data Store Write13 : DataStoreWrite  DataStoreName=AI09
  Data Store Write14 : DataStoreWrite  DataStoreName=AI20
  Data Store Write2 : DataStoreWrite  DataStoreName=AI18
  Data Store Write3 : DataStoreWrite  DataStoreName=AI06
  Data Store Write4 : DataStoreWrite  DataStoreName=AI07
  Data Store Write5 : DataStoreWrite  DataStoreName=AI08
  Data Store Write6 : DataStoreWrite  DataStoreName=AI12
  Data Store Write7 : DataStoreWrite  DataStoreName=AI15
  Data Store Write8 : DataStoreWrite  DataStoreName=AI17
  Data Store Write9 : DataStoreWrite  DataStoreName=AI19
  Data Type Conversion{,1..14} (15 alike) : DataTypeConversion  OutDataTypeStr=single
  Demux : Demux  Outputs=10
  Demux1 : Demux  Outputs=5
  Gain{1,6,8,10,12..14} (7 alike) : Gain  Gain=5/4095
  Gain{2..5,7,11,15} (7 alike) : Gain  Gain=36.6/4095  OutDataTypeStr=single
  Gain9 : Gain  Gain=25.7/4095  OutDataTypeStr=single
  AI : Outport
  wires:
  Demux/4 -> Data Type Conversion3/1
  ADC_Start1/1 -> Demux/1
  Demux/7 -> Data Type Conversion6/1
  Demux1/4 -> Data Type Conversion13/1
  Demux1/3 -> Data Type Conversion12/1
  ADC_Start/1 -> Demux1/1
  Demux1/2 -> Data Type Conversion11/1
  Demux1/5 -> Data Type Conversion14/1
  Demux1/1 -> Data Type Conversion10/1
  Demux/1 -> Data Type Conversion/1
  Demux/3 -> Data Type Conversion2/1
  Demux/2 -> Data Type Conversion1/1
  Demux/5 -> Data Type Conversion4/1
  Demux/8 -> Data Type Conversion7/1
  Demux/9 -> Data Type Conversion8/1
  Demux/10 -> Data Type Conversion9/1
  Demux/6 -> Data Type Conversion5/1
  Data Type Conversion/1 -> Gain6/1
  Gain6/1 -> Data Store Write7/1
  Data Type Conversion1/1 -> Gain7/1
  Data Type Conversion2/1 -> Gain1/1
  Data Type Conversion3/1 -> Gain2/1
  Data Type Conversion4/1 -> Gain8/1
  Data Type Conversion5/1 -> Gain3/1
  Data Type Conversion6/1 -> Gain10/1
  Data Type Conversion7/1 -> Gain12/1
  Data Type Conversion8/1 -> Gain13/1
  Data Type Conversion9/1 -> Gain14/1
  Data Type Conversion10/1 -> Gain4/1
  Data Type Conversion11/1 -> Gain5/1
  Data Type Conversion12/1 -> Gain9/1
  Data Type Conversion13/1 -> Gain11/1
  Data Type Conversion14/1 -> Gain15/1
  Gain7/1 -> Data Store Write2/1
  Gain1/1 -> Data Store Write5/1
  Gain2/1 -> Data Store Write/1
  Gain8/1 -> Data Store Write8/1
  Gain3/1 -> Data Store Write1/1
  Gain10/1 -> Data Store Write3/1
  Gain12/1 -> Data Store Write6/1
  Gain13/1 -> Data Store Write9/1
  Gain14/1 -> Data Store Write4/1
  Gain4/1 -> Data Store Write14/1
  Gain5/1 -> Data Store Write12/1
  Gain9/1 -> Data Store Write10/1
  Gain11/1 -> Data Store Write11/1
  Gain15/1 -> Data Store Write13/1
  Data Store Read/1 -> Bus Creator/1  "AI18"
  Data Store Read1/1 -> Bus Creator/2  "AI11"
  Data Store Read2/1 -> Bus Creator/3  "AI16"
  Data Store Read3/1 -> Bus Creator/4  "AI20"
  Data Store Read4/1 -> Bus Creator/5  "AI05"
  Data Store Read5/1 -> Bus Creator/6  "AI03"
  Data Store Read6/1 -> Bus Creator/7  "AI04"
  Data Store Read7/1 -> Bus Creator/8  "AI09"
  Data Store Read8/1 -> Bus Creator/9  "AI15"
  Data Store Read9/1 -> Bus Creator/10  "AI08"
  Data Store Read10/1 -> Bus Creator/11  "AI17"
  Data Store Read11/1 -> Bus Creator/12  "AI06"
  Data Store Read12/1 -> Bus Creator/13  "AI12"
  Data Store Read13/1 -> Bus Creator/14  "AI19"
  Data Store Read14/1 -> Bus Creator/15  "AI07"
  Bus Creator/1 -> AI/1

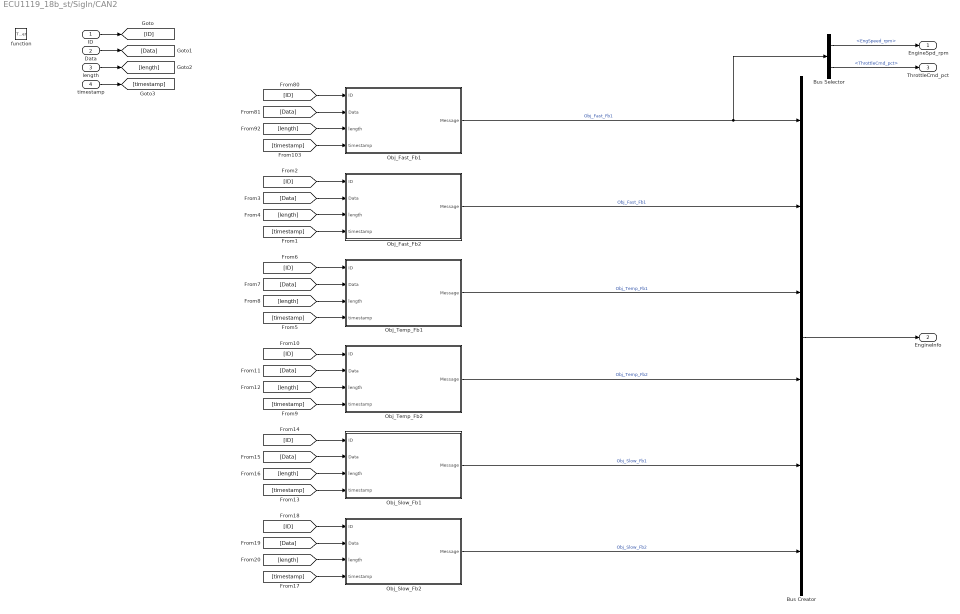
== system ECU1119_18b_st/SigIn/CAN2 ==
  ID : Inport
  Data : Inport  Port=2
  length : Inport  Port=3
  timestamp : Inport  Port=4
  function : TriggerPort  TriggerType=function-call  VariantControl=Variant
  Bus Creator : BusCreator  Inputs=6
  Bus Selector : BusSelector  OutputSignals=EngSpeed_rpm,ThrottleCmd_pct
  Obj_Fast_Fb1 : Subsystem
  Obj_Fast_Fb2 : Subsystem
  Obj_Slow_Fb1 : Subsystem
  Obj_Slow_Fb2 : Subsystem
  Obj_Temp_Fb1 : Subsystem
  Obj_Temp_Fb2 : Subsystem
  EngineSpd_rpm : Outport
  EngineInfo : Outport  Port=2
  ThrottleCmd_pct : Outport  Port=3
  wires:
  Obj_Fast_Fb1/1(Message) -> Bus Selector/1, Bus Creator/1  "Obj_Fast_Fb1"
  [timestamp] -> Obj_Fast_Fb1/4(timestamp)
  [length] -> Obj_Fast_Fb1/3(length)
  [Data] -> Obj_Fast_Fb1/2(Data)
  [ID] -> Obj_Fast_Fb1/1(ID)
  length/1 -> [length]
  ID/1 -> [ID]
  timestamp/1 -> [timestamp]
  Data/1 -> [Data]
  [ID] -> Obj_Fast_Fb2/1(ID)
  [Data] -> Obj_Fast_Fb2/2(Data)
  [length] -> Obj_Fast_Fb2/3(length)
  [timestamp] -> Obj_Fast_Fb2/4(timestamp)
  Obj_Fast_Fb2/1(Message) -> Bus Creator/2  "Obj_Fast_Fb1"
  Obj_Temp_Fb1/1(Message) -> Bus Creator/3  "Obj_Temp_Fb1"
  [timestamp] -> Obj_Temp_Fb1/4(timestamp)
  [length] -> Obj_Temp_Fb1/3(length)
  [Data] -> Obj_Temp_Fb1/2(Data)
  [ID] -> Obj_Temp_Fb1/1(ID)
  [ID] -> Obj_Temp_Fb2/1(ID)
  [Data] -> Obj_Temp_Fb2/2(Data)
  [length] -> Obj_Temp_Fb2/3(length)
  [timestamp] -> Obj_Temp_Fb2/4(timestamp)
  Obj_Temp_Fb2/1(Message) -> Bus Creator/4  "Obj_Temp_Fb2"
  [ID] -> Obj_Slow_Fb1/1(ID)
  [Data] -> Obj_Slow_Fb1/2(Data)
  [length] -> Obj_Slow_Fb1/3(length)
  [timestamp] -> Obj_Slow_Fb1/4(timestamp)
  Obj_Slow_Fb1/1(Message) -> Bus Creator/5  "Obj_Slow_Fb1"
  Obj_Slow_Fb2/1(Message) -> Bus Creator/6  "Obj_Slow_Fb2"
  [length] -> Obj_Slow_Fb2/3(length)
  [Data] -> Obj_Slow_Fb2/2(Data)
  [ID] -> Obj_Slow_Fb2/1(ID)
  [timestamp] -> Obj_Slow_Fb2/4(timestamp)
  Bus Selector/1 -> EngineSpd_rpm/1  "<EngSpeed_rpm>"
  Bus Selector/2 -> ThrottleCmd_pct/1  "<ThrottleCmd_pct>"
  Bus Creator/1 -> EngineInfo/1

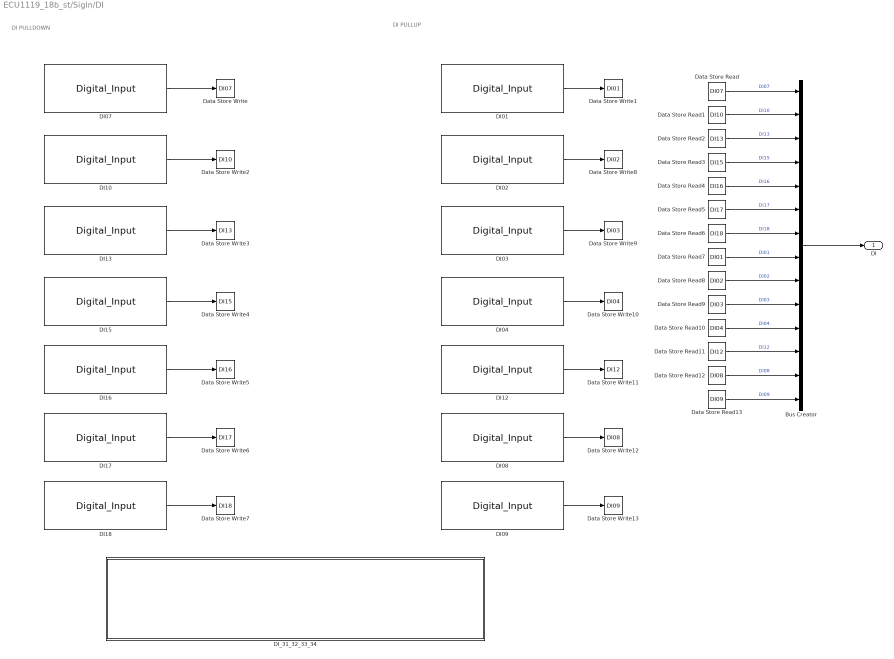
== system ECU1119_18b_st/SigIn/DI ==
  note: DI PULLDOWN
  note: DI PULLUP
  Bus Creator : BusCreator  Inputs=14
  DI01 : mbd_mpc574x_ec_toolbox/GPIO Blocks/Digital_Input  gpio_pin=PTG5: [SIUL2_GPIO101 | General Purpose IO PG[5]]  pull_resistor=None
      settings: SourceProductName=NXP Model-Based Design Toolbox for MPC57xx MCUs
  DI02 : mbd_mpc574x_ec_toolbox/GPIO Blocks/Digital_Input  gpio_pin=PTG9: [SIUL2_GPIO105 | General Purpose IO PG[9]]  pull_resistor=None
      settings: SourceProductName=NXP Model-Based Design Toolbox for MPC57xx MCUs
  DI03 : mbd_mpc574x_ec_toolbox/GPIO Blocks/Digital_Input  gpio_pin=PTC11: [SIUL2_GPIO43 | General Purpose IO PC[11]]  pull_resistor=None
      settings: SourceProductName=NXP Model-Based Design Toolbox for MPC57xx MCUs
  DI04 : mbd_mpc574x_ec_toolbox/GPIO Blocks/Digital_Input  gpio_pin=PTA9: [SIUL2_GPIO9 | General Purpose IO PA[9]]  pull_resistor=None
      settings: SourceProductName=NXP Model-Based Design Toolbox for MPC57xx MCUs
  DI07 : mbd_mpc574x_ec_toolbox/GPIO Blocks/Digital_Input  gpio_pin=PTA0: [SIUL2_GPIO0 | General Purpose IO PA[0]]  pull_resistor=None
      settings: SourceProductName=NXP Model-Based Design Toolbox for MPC57xx MCUs
  DI08 : mbd_mpc574x_ec_toolbox/GPIO Blocks/Digital_Input  gpio_pin=PTD11: [SIUL2_GPIO59 | General Purpose IO PD[11]]  pull_resistor=None
      settings: SourceProductName=NXP Model-Based Design Toolbox for MPC57xx MCUs
  DI09 : mbd_mpc574x_ec_toolbox/GPIO Blocks/Digital_Input  gpio_pin=PTG6: [SIUL2_GPIO102 | General Purpose IO PG[6]]  pull_resistor=None
      settings: SourceProductName=NXP Model-Based Design Toolbox for MPC57xx MCUs
  DI10 : mbd_mpc574x_ec_toolbox/GPIO Blocks/Digital_Input  gpio_pin=PTG2: [SIUL2_GPIO98 | General Purpose IO PG[2]]  pull_resistor=None
      settings: SourceProductName=NXP Model-Based Design Toolbox for MPC57xx MCUs
  DI12 : mbd_mpc574x_ec_toolbox/GPIO Blocks/Digital_Input  gpio_pin=PTF13: [SIUL2_GPIO93 | General Purpose IO PF[13]]  pull_resistor=None
      settings: SourceProductName=NXP Model-Based Design Toolbox for MPC57xx MCUs
  DI13 : mbd_mpc574x_ec_toolbox/GPIO Blocks/Digital_Input  gpio_pin=PTG4: [SIUL2_GPIO100 | General Purpose IO PG[4]]  pull_resistor=None
      settings: SourceProductName=NXP Model-Based Design Toolbox for MPC57xx MCUs
  DI15 : mbd_mpc574x_ec_toolbox/GPIO Blocks/Digital_Input  gpio_pin=PTF12: [SIUL2_GPIO92 | General Purpose IO PF[12]]  pull_resistor=None
      settings: SourceProductName=NXP Model-Based Design Toolbox for MPC57xx MCUs
  DI16 : mbd_mpc574x_ec_toolbox/GPIO Blocks/Digital_Input  gpio_pin=PTG7: [SIUL2_GPIO103 | General Purpose IO PG[7]]  pull_resistor=None
      settings: SourceProductName=NXP Model-Based Design Toolbox for MPC57xx MCUs
  DI17 : mbd_mpc574x_ec_toolbox/GPIO Blocks/Digital_Input  gpio_pin=PTD10: [SIUL2_GPIO58 | General Purpose IO PD[10]]  pull_resistor=None
      settings: SourceProductName=NXP Model-Based Design Toolbox for MPC57xx MCUs
  DI18 : mbd_mpc574x_ec_toolbox/GPIO Blocks/Digital_Input  gpio_pin=PTG10: [SIUL2_GPIO106 | General Purpose IO PG[10]]  pull_resistor=None
      settings: SourceProductName=NXP Model-Based Design Toolbox for MPC57xx MCUs
  DI_31_32_33_34 : Subsystem
  Data Store Read : DataStoreRead  DataStoreName=DI07
  Data Store Read1 : DataStoreRead  DataStoreName=DI10
  Data Store Read10 : DataStoreRead  DataStoreName=DI04
  Data Store Read11 : DataStoreRead  DataStoreName=DI12
  Data Store Read12 : DataStoreRead  DataStoreName=DI08
  Data Store Read13 : DataStoreRead  DataStoreName=DI09
  Data Store Read2 : DataStoreRead  DataStoreName=DI13
  Data Store Read3 : DataStoreRead  DataStoreName=DI15
  Data Store Read4 : DataStoreRead  DataStoreName=DI16
  Data Store Read5 : DataStoreRead  DataStoreName=DI17
  Data Store Read6 : DataStoreRead  DataStoreName=DI18
  Data Store Read7 : DataStoreRead  DataStoreName=DI01
  Data Store Read8 : DataStoreRead  DataStoreName=DI02
  Data Store Read9 : DataStoreRead  DataStoreName=DI03
  Data Store Write : DataStoreWrite  DataStoreName=DI07
  Data Store Write1 : DataStoreWrite  DataStoreName=DI01
  Data Store Write10 : DataStoreWrite  DataStoreName=DI04
  Data Store Write11 : DataStoreWrite  DataStoreName=DI12
  Data Store Write12 : DataStoreWrite  DataStoreName=DI08
  Data Store Write13 : DataStoreWrite  DataStoreName=DI09
  Data Store Write2 : DataStoreWrite  DataStoreName=DI10
  Data Store Write3 : DataStoreWrite  DataStoreName=DI13
  Data Store Write4 : DataStoreWrite  DataStoreName=DI15
  Data Store Write5 : DataStoreWrite  DataStoreName=DI16
  Data Store Write6 : DataStoreWrite  DataStoreName=DI17
  Data Store Write7 : DataStoreWrite  DataStoreName=DI18
  Data Store Write8 : DataStoreWrite  DataStoreName=DI02
  Data Store Write9 : DataStoreWrite  DataStoreName=DI03
  DI : Outport
  wires:
  DI07/1 -> Data Store Write/1
  DI01/1 -> Data Store Write1/1
  DI10/1 -> Data Store Write2/1
  DI13/1 -> Data Store Write3/1
  DI15/1 -> Data Store Write4/1
  DI17/1 -> Data Store Write6/1
  DI16/1 -> Data Store Write5/1
  DI18/1 -> Data Store Write7/1
  DI09/1 -> Data Store Write13/1
  DI08/1 -> Data Store Write12/1
  DI12/1 -> Data Store Write11/1
  DI04/1 -> Data Store Write10/1
  DI02/1 -> Data Store Write8/1
  DI03/1 -> Data Store Write9/1
  Data Store Read/1 -> Bus Creator/1  "DI07"
  Data Store Read1/1 -> Bus Creator/2  "DI10"
  Data Store Read2/1 -> Bus Creator/3  "DI13"
  Data Store Read3/1 -> Bus Creator/4  "DI15"
  Data Store Read4/1 -> Bus Creator/5  "DI16"
  Data Store Read5/1 -> Bus Creator/6  "DI17"
  Data Store Read6/1 -> Bus Creator/7  "DI18"
  Data Store Read7/1 -> Bus Creator/8  "DI01"
  Data Store Read8/1 -> Bus Creator/9  "DI02"
  Data Store Read9/1 -> Bus Creator/10  "DI03"
  Data Store Read10/1 -> Bus Creator/11  "DI04"
  Data Store Read11/1 -> Bus Creator/12  "DI12"
  Data Store Read12/1 -> Bus Creator/13  "DI08"
  Data Store Read13/1 -> Bus Creator/14  "DI09"
  Bus Creator/1 -> DI/1
